simulink model "generic_src"  (Simulink 10.3)
settings: Solver=ode45  StartTime=0.0  StopTime=inf  RelTol=1e-3  EnableMultiTasking=on
undefined symbols (not defined in the file or in its folder): Area_Front, Area_Rear, ay_max_off, ay_max_on, ay_per_mu_max_off, ay_per_mu_max_on, Brake_ratio, brake_valve_ctrl_kP, cat1mode1_higher, cat1mode1_lower, cat1mode2_higher, cat1mode2_lower, cat1mode3_higher, cat1mode3_lower, cat2mode1_higher, cat2mode1_lower, cat2mode2_higher, cat2mode2_lower, cat2mode3_higher, cat2mode3_lower, delta_vel, diff_lock_fac, diff_lock_off, diff_lock_on, ESP_ctrl_kD, ESP_ctrl_kI, ESP_ctrl_kP, ESP_ctrl_restore_kI, ESP_min_throttle_fac, f_ax, f_slip, g, higherlimit_highvel, higherlimit_lowvel, highervel_fac, highervelocity_fac, InitialConditionForIntegrator, limit_acc, limit_selectlow, limit_starting, limit_vdiff, locktime_throttle, lowerlimit_highvel, lowerlimit_lowvel, lowervel_fac, lowervelocity_fac, min_throttle, MPS2KMPH, MSR_ctrl_kD, MSR_ctrl_kI, MSR_ctrl_kP, MSR_min_throttle_fac, PID_kP_sideslip, PID_kP_yawrate, RADpS2RpM, rBrake, RpM2RADpS, SH_SL_switch, sideslip_vel_corr, sidesplip_deviation_max ... (+35)
libraries: CarMaker4SL x136, simulink x55, simulink_extras x6
(part 8 of 9)

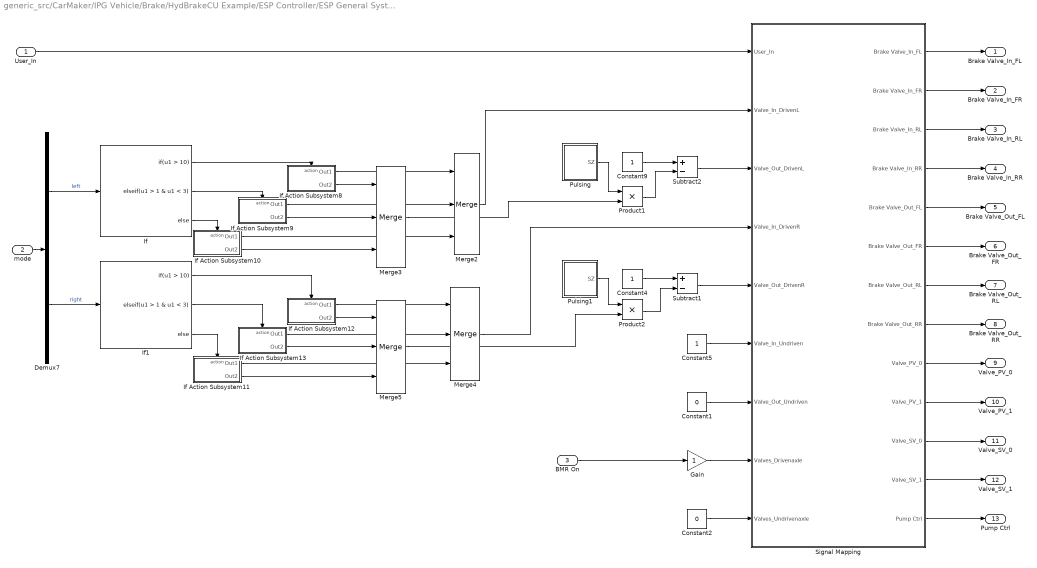
== system generic_src/CarMaker/IPG Vehicle/Brake/HydBrakeCU Example/ESP Controller/ESP General System/ASR/BMR ECU/BMR Controller ==
  User_In : Inport
  mode : Inport  Port=2
  BMR On : Inport  Port=3
  Constant1 : Constant  Value=0
  Constant2 : Constant  Value=0
  Constant4 : Constant
  Constant5 : Constant
  Constant9 : Constant
  Demux7 : Demux  Outputs=2
  Gain : Gain
  If : If  IfExpression=u1 > 10  ElseIfExpressions=u1 > 1 & u1 < 3
  If Action Subsystem10 : Subsystem  TreatAsAtomicUnit=on
  If Action Subsystem11 : Subsystem  TreatAsAtomicUnit=on
  If Action Subsystem12 : Subsystem  TreatAsAtomicUnit=on
  If Action Subsystem13 : Subsystem  TreatAsAtomicUnit=on
  If Action Subsystem8 : Subsystem  TreatAsAtomicUnit=on
  If Action Subsystem9 : Subsystem  TreatAsAtomicUnit=on
  If1 : If  IfExpression=u1 > 10  ElseIfExpressions=u1 > 1 & u1 < 3
  Merge{2..5} (4 alike) : Merge  Inputs=3
  Product1 : Product  RndMeth=Zero
  Product2 : Product  RndMeth=Zero
  Pulsing : Subsystem
  Pulsing1 : Subsystem
  Signal Mapping : Subsystem
  Subtract1 : Sum  Inputs=+-
  Subtract2 : Sum  Inputs=+-
  Brake Valve_In_FL : Outport  VectorParamsAs1DForOutWhenUnconnected=off
  Brake Valve_In_FR : Outport  Port=2  VectorParamsAs1DForOutWhenUnconnected=off
  Brake Valve_In_RL : Outport  Port=3  VectorParamsAs1DForOutWhenUnconnected=off
  Brake Valve_In_RR : Outport  Port=4  VectorParamsAs1DForOutWhenUnconnected=off
  Brake Valve_Out_FL : Outport  Port=5  VectorParamsAs1DForOutWhenUnconnected=off
  Brake Valve_Out_FR : Outport  Port=6  VectorParamsAs1DForOutWhenUnconnected=off
  Brake Valve_Out_RL : Outport  Port=7  VectorParamsAs1DForOutWhenUnconnected=off
  Brake Valve_Out_RR : Outport  Port=8  VectorParamsAs1DForOutWhenUnconnected=off
  Valve_PV_0 : Outport  Port=9  VectorParamsAs1DForOutWhenUnconnected=off
  Valve_PV_1 : Outport  Port=10  VectorParamsAs1DForOutWhenUnconnected=off
  Valve_SV_0 : Outport  Port=11  VectorParamsAs1DForOutWhenUnconnected=off
  Valve_SV_1 : Outport  Port=12  VectorParamsAs1DForOutWhenUnconnected=off
  Pump Ctrl : Outport  Port=13  VectorParamsAs1DForOutWhenUnconnected=off
  wires:
  Demux7/1 -> If/1  "left"
  If/1 -> If Action Subsystem8/Action
  If/2 -> If Action Subsystem9/Action
  If/3 -> If Action Subsystem10/Action
  If Action Subsystem8/1(Out1) -> Merge2/1
  If Action Subsystem9/1(Out1) -> Merge2/2
  If Action Subsystem10/1(Out1) -> Merge2/3
  If Action Subsystem8/2(Out2) -> Merge3/1
  If Action Subsystem9/2(Out2) -> Merge3/2
  If Action Subsystem10/2(Out2) -> Merge3/3
  If1/1 -> If Action Subsystem12/Action
  If1/2 -> If Action Subsystem13/Action
  If1/3 -> If Action Subsystem11/Action
  If Action Subsystem12/1(Out1) -> Merge4/1
  If Action Subsystem13/1(Out1) -> Merge4/2
  If Action Subsystem11/1(Out1) -> Merge4/3
  If Action Subsystem12/2(Out2) -> Merge5/1
  If Action Subsystem13/2(Out2) -> Merge5/2
  If Action Subsystem11/2(Out2) -> Merge5/3
  Demux7/2 -> If1/1  "right"
  Merge3/1 -> Product1/2
  Merge5/1 -> Product2/2
  Constant4/1 -> Subtract1/1
  Product2/1 -> Subtract1/2
  Constant9/1 -> Subtract2/1
  Product1/1 -> Subtract2/2
  BMR On/1 -> Gain/1
  mode/1 -> Demux7/1
  Merge2/1 -> Signal Mapping/2(Valve_In_DrivenL)
  Merge4/1 -> Signal Mapping/4(Valve_In_DrivenR)
  Constant5/1 -> Signal Mapping/6(Valve_In_Undriven)
  Constant1/1 -> Signal Mapping/7(Valve_Out_Undriven)
  Gain/1 -> Signal Mapping/8(Valves_Drivenaxle)
  Constant2/1 -> Signal Mapping/9(Valves_Undrivenaxle)
  Signal Mapping/1(Brake Valve_In_FL) -> Brake Valve_In_FL/1
  Signal Mapping/2(Brake Valve_In_FR) -> Brake Valve_In_FR/1
  Signal Mapping/3(Brake Valve_In_RL) -> Brake Valve_In_RL/1
  Signal Mapping/4(Brake Valve_In_RR) -> Brake Valve_In_RR/1
  Signal Mapping/5(Brake Valve_Out_FL) -> Brake Valve_Out_FL/1
  Signal Mapping/6(Brake Valve_Out_FR) -> Brake Valve_Out_FR/1
  Signal Mapping/7(Brake Valve_Out_RL) -> Brake Valve_Out_RL/1
  Signal Mapping/8(Brake Valve_Out_RR) -> Brake Valve_Out_RR/1
  Signal Mapping/9(Valve_PV_0) -> Valve_PV_0/1
  Signal Mapping/10(Valve_PV_1) -> Valve_PV_1/1
  Signal Mapping/11(Valve_SV_0) -> Valve_SV_0/1
  Signal Mapping/12(Valve_SV_1) -> Valve_SV_1/1
  Signal Mapping/13(Pump Ctrl) -> Pump Ctrl/1
  User_In/1 -> Signal Mapping/1(User_In)
  Subtract1/1 -> Signal Mapping/5(Valve_Out_DrivenR)
  Subtract2/1 -> Signal Mapping/3(Valve_Out_DrivenL)
  Pulsing1/1(SZ) -> Product2/1
  Pulsing/1(SZ) -> Product1/1

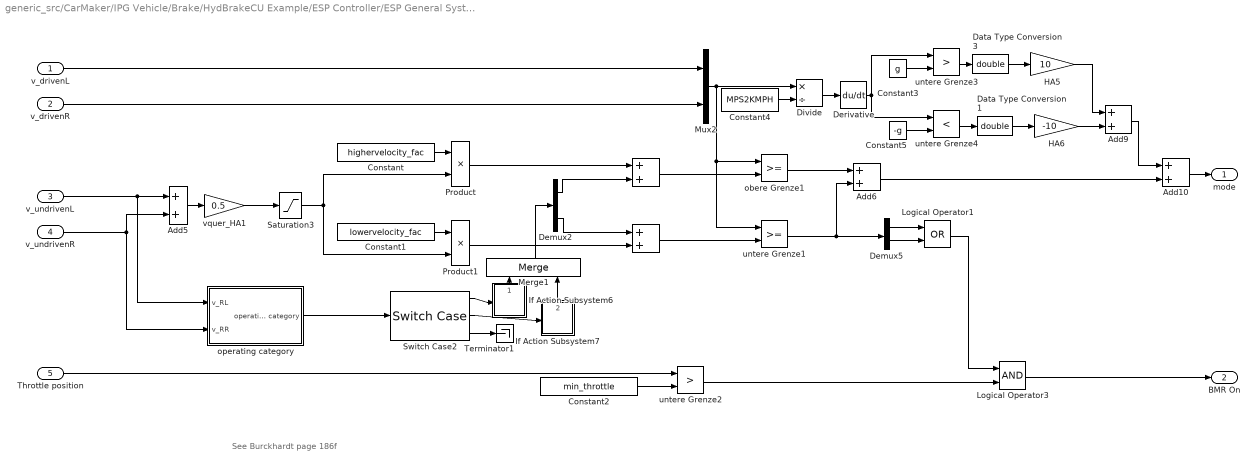
== system generic_src/CarMaker/IPG Vehicle/Brake/HydBrakeCU Example/ESP Controller/ESP General System/ASR/BMR ECU/BMR logic ==
  note: See Burckhardt page 186f
  v_drivenL : Inport
  v_drivenR : Inport  Port=2
  v_undrivenL : Inport  Port=3
  v_undrivenR : Inport  Port=4
  Throttle position : Inport  Port=5
  " " : Sum
  "   " : Sum
  Add{5..6,9..10} (4 alike) : Sum
  Constant : Constant  Value=highervelocity_fac
  Constant1 : Constant  Value=lowervelocity_fac
  Constant2 : Constant  Value=min_throttle
  Constant3 : Constant  Value=g
  Constant4 : Constant  Value=MPS2KMPH
  Constant5 : Constant  Value=-g
  Data Type Conversion1 : DataTypeConversion  OutDataTypeStr=double
  Data Type Conversion3 : DataTypeConversion  OutDataTypeStr=double
  Demux2 : Demux  Outputs=2
  Demux5 : Demux  Outputs=2
  Derivative : Derivative
  Divide : Product  Inputs=*/
  HA5 : Gain  Gain=10
  HA6 : Gain  Gain=-10
  If Action Subsystem6 : Subsystem  TreatAsAtomicUnit=on
  If Action Subsystem7 : Subsystem  TreatAsAtomicUnit=on
  Logical Operator1 : Logic  Operator=OR  AllPortsSameDT=off
  Logical Operator3 : Logic  AllPortsSameDT=off
  Merge1 : Merge
  Mux2 : Mux  Inputs=2
  Product : Product  RndMeth=Zero
  Product1 : Product  RndMeth=Zero
  Saturation3 : Saturate  UpperLimit=inf  LowerLimit=1
  Switch Case2 : SwitchCase  CaseConditions={1,2}
  Terminator1 : Terminator
  obere Grenze1 : RelationalOperator  OutDataTypeStr=boolean  RndMeth=Nearest
  operating category : Subsystem
  untere Grenze1 : RelationalOperator  OutDataTypeStr=boolean  RndMeth=Nearest
  untere Grenze2 : RelationalOperator  Operator=>  RndMeth=Nearest
  untere Grenze3 : RelationalOperator  Operator=>  RndMeth=Nearest
  untere Grenze4 : RelationalOperator  Operator=<  RndMeth=Nearest
  vquer_HA1 : Gain  Gain=0.5
  mode : Outport  VectorParamsAs1DForOutWhenUnconnected=off
  BMR On : Outport  Port=2  VectorParamsAs1DForOutWhenUnconnected=off
  wires:
  Switch Case2/3 -> Terminator1/1
  operating category/1(operating category) -> Switch Case2/1
  Switch Case2/1 -> If Action Subsystem6/Action
  Switch Case2/2 -> If Action Subsystem7/Action
  Merge1/1 -> Demux2/1
  If Action Subsystem6/1(1) -> Merge1/1
  If Action Subsystem7/1(2) -> Merge1/2
  Demux2/1 -> "   "/2
  Add5/1 -> vquer_HA1/1
  vquer_HA1/1 -> Saturation3/1
  Saturation3/1 -> Product1/2, Product/2
  Product/1 -> "   "/1
  Product1/1 -> " "/2
  Demux2/2 -> " "/1
  "   "/1 -> obere Grenze1/2
  obere Grenze1/1 -> Add6/1
  untere Grenze1/1 -> Add6/2, Demux5/1
  untere Grenze3/1 -> Data Type Conversion3/1
  untere Grenze4/1 -> Data Type Conversion1/1
  HA5/1 -> Add9/1
  HA6/1 -> Add9/2
  Data Type Conversion3/1 -> HA5/1
  Data Type Conversion1/1 -> HA6/1
  Derivative/1 -> untere Grenze4/1, untere Grenze3/1
  Add6/1 -> Add10/2
  Divide/1 -> Derivative/1
  Add9/1 -> Add10/1
  Add10/1 -> mode/1
  Demux5/1 -> Logical Operator1/1
  Demux5/2 -> Logical Operator1/2
  Logical Operator3/1 -> BMR On/1
  Throttle position/1 -> untere Grenze2/1
  Logical Operator1/1 -> Logical Operator3/1
  untere Grenze2/1 -> Logical Operator3/2
  v_undrivenL/1 -> operating category/1(v_RL), Add5/1
  v_undrivenR/1 -> Add5/2, operating category/2(v_RR)
  Constant/1 -> Product/1
  Constant1/1 -> Product1/1
  Constant2/1 -> untere Grenze2/2
  Constant4/1 -> Divide/2
  Constant3/1 -> untere Grenze3/2
  Constant5/1 -> untere Grenze4/2
  " "/1 -> untere Grenze1/2
  Mux2/1 -> Divide/1, obere Grenze1/1, untere Grenze1/1
  v_drivenR/1 -> Mux2/2
  v_drivenL/1 -> Mux2/1

== system generic_src/CarMaker/IPG Vehicle/Brake/HydBrakeCU Example/ESP Controller/ESP General System/ASR/BMR ECU/Differential Lock ==
  User_In : Inport
  v_DrivenL : Inport  Port=2
  v_DrivenR : Inport  Port=3
  Abs : Abs
  Add1 : Sum  Inputs=+-
  Bus Selector1 : BusSelector  OutputSignals=User_DiffLock.User_DiffLock_Trq,User_DiffLock.User_DiffLock_on
  Bus Selector2 : BusSelector  OutputSignals=User_Drive
  Constant : Constant  Value=0
  Constant1 : Constant  Value=0
  Constant2 : Constant  Value=diff_lock_fac
  Demux : Demux  Outputs=2
  Mux : Mux  Inputs=2
  Mux1 : Mux  Inputs=2
  Mux2 : Mux  Inputs=2
  Product : Product  RndMeth=Zero
  Relay : Relay  OnSwitchValue=diff_lock_on  OffSwitchValue=diff_lock_off
  Switch1 : Switch  Criteria=u2 > Threshold
  Switch2 : Switch  Criteria=u2 > Threshold  Threshold=1.5
  Switch3 : Switch  Criteria=u2 > Threshold  Threshold=2.5
  Transfer Fcn : TransferFcn  Denominator=[0.1 1]
  FrontDiff_Torque : Outport  VectorParamsAs1DForOutWhenUnconnected=off
  RearDiff_Torque : Outport  Port=2  VectorParamsAs1DForOutWhenUnconnected=off
  wires:
  Abs/1 -> Relay/1
  Relay/1 -> Product/1
  Add1/1 -> Abs/1
  Product/1 -> Transfer Fcn/1
  v_DrivenL/1 -> Add1/1
  v_DrivenR/1 -> Add1/2
  User_In/1 -> Bus Selector2/1, Bus Selector1/1
  Bus Selector2/1 -> Switch2/2, Switch3/2  "<User_Drive>"
  Demux/1 -> FrontDiff_Torque/1
  Demux/2 -> RearDiff_Torque/1
  Switch3/1 -> Demux/1
  Transfer Fcn/1 -> Switch1/3
  Mux/1 -> Switch3/1
  Constant/1 -> Mux1/1
  Mux1/1 -> Switch2/1
  Switch2/1 -> Switch3/3
  Constant1/1 -> Mux2/2
  Mux2/1 -> Switch2/3
  Bus Selector1/2 -> Switch1/2  "<User_DiffLock_on>"
  Bus Selector1/1 -> Switch1/1  "<User_DiffLock_Trq>"
  Switch1/1 -> Mux2/1, Mux1/2, Mux/1, Mux/2
  Constant2/1 -> Product/2

== system generic_src/CarMaker/IPG Vehicle/Brake/HydBrakeCU Example/ESP Controller/ESP General System/ASR/BMR ECU/Signal Mapping ==
  User_In : Inport
  WheelVelocity : Inport  Port=2
  Ideal_In : Inport  Port=3
  Bus Selector1 : BusSelector  OutputSignals=Ideal_Velocity.Ideal_Velocity
  Bus Selector2 : BusSelector  OutputSignals=User_Drive
  Demux1 : Demux
  Demux2 : Demux
  Mux1 : Mux
  Mux2 : Mux
  Mux3 : Mux
  Switch2 : Switch  Criteria=u2 > Threshold  Threshold=1.5
  Switch3 : Switch  Criteria=u2 > Threshold  Threshold=2.5
  v_DrivenL : Outport  VectorParamsAs1DForOutWhenUnconnected=off
  v_DrivenR : Outport  Port=2  VectorParamsAs1DForOutWhenUnconnected=off
  v_UndrivenL : Outport  Port=3  VectorParamsAs1DForOutWhenUnconnected=off
  v_UndrivenR : Outport  Port=4  VectorParamsAs1DForOutWhenUnconnected=off
  wires:
  WheelVelocity/1 -> Demux1/1
  User_In/1 -> Bus Selector2/1
  Bus Selector2/1 -> Switch3/2, Switch2/2  "<User_Drive>"
  Bus Selector1/1 -> Mux3/3, Mux3/4  "<Ideal_Velocity>"
  Mux3/1 -> Switch3/1
  Switch2/1 -> Switch3/3
  Switch3/1 -> Demux2/1
  Demux1/1 -> Mux1/1, Mux3/1, Mux2/3  "v_FL"
  Demux1/2 -> Mux1/2, Mux2/4, Mux3/2  "v_FR"
  Demux1/3 -> Mux1/3, Mux2/1
  Demux1/4 -> Mux1/4, Mux2/2
  Mux1/1 -> Switch2/3
  Mux2/1 -> Switch2/1
  Demux2/1 -> v_DrivenL/1
  Demux2/2 -> v_DrivenR/1
  Demux2/3 -> v_UndrivenL/1
  Demux2/4 -> v_UndrivenR/1
  Ideal_In/1 -> Bus Selector1/1

== system generic_src/CarMaker/IPG Vehicle/Brake/HydBrakeCU Example/ESP Controller/ESP General System/ASR/MSR ECU/MSR logic ==
  v_drivenL : Inport
  v_drivenR : Inport  Port=2
  v_undrivenL : Inport  Port=3
  v_undrivenR : Inport  Port=4
  " " : Gain  Gain=0.5
  "   " : Gain  Gain=0.5
  Add{,1..4} (5 alike) : Sum
  Compare To Zero : simulink/Logic and Bit Operations/Compare To Zero  relop===  OutDataTypeStr=uint8
  Constant : Constant  Value=highervel_fac
  Constant1 : Constant  Value=lowervel_fac
  Demux1 : Demux  Outputs=2
  If Action Subsystem : Subsystem  TreatAsAtomicUnit=on
  If Action Subsystem1 : Subsystem  TreatAsAtomicUnit=on
  If Action Subsystem2 : Subsystem  TreatAsAtomicUnit=on
  If Action Subsystem3 : Subsystem  TreatAsAtomicUnit=on
  If Action Subsystem4 : Subsystem  TreatAsAtomicUnit=on
  If Action Subsystem5 : Subsystem  TreatAsAtomicUnit=on
  Logical Operator : Logic  AllPortsSameDT=off  OutDataTypeStr=boolean
  Merge : Merge  Inputs=6
  Product : Product  RndMeth=Zero
  Product1 : Product  RndMeth=Zero
  Saturation1 : Saturate  UpperLimit=inf  LowerLimit=1
  Saturation2 : Saturate  UpperLimit=inf  LowerLimit=1
  Subtract : Sum  Inputs=+-
  Subtract3 : Sum  Inputs=+-
  Switch Case1 : SwitchCase  CaseConditions={11,12,13,21,22,23}
  Terminator : Terminator
  lower bound : RelationalOperator  OutDataTypeStr=boolean  RndMeth=Nearest
  operating category : Subsystem
  operating mode : Subsystem
  upper bound : RelationalOperator  OutDataTypeStr=boolean  RndMeth=Nearest
  Pseudo_slip : Outport  VectorParamsAs1DForOutWhenUnconnected=off
  reduce torque : Outport  Port=2  VectorParamsAs1DForOutWhenUnconnected=off
  hold torque : Outport  Port=3  VectorParamsAs1DForOutWhenUnconnected=off
  wires:
  Add1/1 -> " "/1
  Add/1 -> "   "/1
  "   "/1 -> Saturation2/1
  " "/1 -> Saturation1/1
  Product/1 -> Add4/1
  operating mode/1(mode) -> Add3/1
  operating category/1(category) -> Add3/2
  Add3/1 -> Switch Case1/1
  Switch Case1/1 -> If Action Subsystem/Action
  Merge/1 -> Demux1/1
  Switch Case1/2 -> If Action Subsystem1/Action
  Switch Case1/3 -> If Action Subsystem2/Action
  Switch Case1/4 -> If Action Subsystem3/Action
  Switch Case1/5 -> If Action Subsystem4/Action
  Switch Case1/6 -> If Action Subsystem5/Action
  If Action Subsystem/1(1.1) -> Merge/1
  If Action Subsystem1/1(1.2) -> Merge/2
  If Action Subsystem2/1(1.3) -> Merge/3
  If Action Subsystem3/1(2.1) -> Merge/4
  If Action Subsystem4/1(2.2) -> Merge/5
  If Action Subsystem5/1(2.3) -> Merge/6
  Switch Case1/7 -> Terminator/1
  Demux1/1 -> Add4/2
  Add2/1 -> lower bound/2, Subtract3/2
  upper bound/1 -> reduce torque/1, Compare To Zero/1  "reduce moment flag"
  lower bound/1 -> Logical Operator/2
  Compare To Zero/1 -> Logical Operator/1
  Logical Operator/1 -> hold torque/1  "hold moment flag"
  Subtract/1 -> upper bound/1, lower bound/1, Subtract3/1
  Saturation1/1 -> Subtract/1
  Saturation2/1 -> Product1/1, Subtract/2, Product/2
  Add4/1 -> upper bound/2
  Subtract3/1 -> Pseudo_slip/1
  Demux1/2 -> Add2/1
  Product1/1 -> Add2/2
  v_drivenL/1 -> operating category/1(v_drivenL), Add1/1
  v_drivenR/1 -> operating category/2(v_drivenR), Add1/2
  v_undrivenR/1 -> operating category/4(v_undrivenR), operating mode/2(v_undrivenR), Add/2
  v_undrivenL/1 -> operating category/3(v_undrivenL), operating mode/1(v_undrivenL), Add/1
  Constant/1 -> Product/1
  Constant1/1 -> Product1/2

== system generic_src/CarMaker/IPG Vehicle/Brake/HydBrakeCU Example/ESP Controller/ESP General System/ASR/MSR ECU/MSR/Gas Controller ==
  Throttle_position : Inport
  Pseudo_Slip : Inport  Port=2
  close Gas : Inport  Port=3
  hold Gas : Inport  Port=4
  Compare To Zero : simulink/Logic and Bit Operations/Compare To Zero  relop===  OutDataTypeStr=uint8
  Constant1 : Constant  Value=MSR_min_throttle_fac
  Constant2 : Constant  Value=min_throttle
  Data Type Conversion2 : DataTypeConversion
  Enabled Subsystem : Subsystem  TreatAsAtomicUnit=on
  Logical Operator : Logic  Operator=OR  AllPortsSameDT=off
  Logical Operator1 : Logic  AllPortsSameDT=off
  PID Controller : Subsystem
  Product2 : Product  SaturateOnIntegerOverflow=on  OutDataTypeStr=Inherit: Same as first input
  Saturation Dynamic : simulink/Discontinuities/Saturation Dynamic  OutMin=[]  OutMax=[]  OutDataTypeStr=Inherit: Same as second input  OutDataType=sfix(16)  OutScaling=2^-10  DoSatur=off
  Subtract : Sum  Inputs=-+
  Switch1 : Switch  Criteria=u2 > Threshold  Threshold=0.5
  Switch3 : Switch  Criteria=u2 > Threshold
  untere Grenze2 : RelationalOperator  Operator=>  RndMeth=Nearest
  vquer_VA1 : Gain
  MSR_On : Outport  VectorParamsAs1DForOutWhenUnconnected=off
  Gas_Out : Outport  Port=2  VectorParamsAs1DForOutWhenUnconnected=off
  wires:
  hold Gas/1 -> Enabled Subsystem/Trigger, Logical Operator/2, Switch1/2
  Switch3/1 -> Switch1/3, Enabled Subsystem/1(In1)
  Compare To Zero/1 -> Data Type Conversion2/1
  close Gas/1 -> Logical Operator/1, Compare To Zero/1, Switch3/2
  Data Type Conversion2/1 -> PID Controller/2(RESET)
  Enabled Subsystem/1(Out1) -> Switch1/1
  Switch1/1 -> Gas_Out/1
  Throttle_position/1 -> Switch3/3, Product2/1, vquer_VA1/1, Subtract/2, untere Grenze2/1
  PID Controller/1(y) -> Subtract/1
  Pseudo_Slip/1 -> PID Controller/1(u)
  Saturation Dynamic/1 -> Switch3/1
  vquer_VA1/1 -> Saturation Dynamic/1
  Product2/1 -> Saturation Dynamic/3
  Subtract/1 -> Saturation Dynamic/2
  Constant1/1 -> Product2/2
  Constant2/1 -> untere Grenze2/2
  untere Grenze2/1 -> Logical Operator1/2
  Logical Operator/1 -> Logical Operator1/1
  Logical Operator1/1 -> MSR_On/1

== system generic_src/CarMaker/IPG Vehicle/Brake/HydBrakeCU Example/ESP Controller/ESP General System/ASR/MSR ECU/Signal Mapping ==
  WheelVelocity : Inport
  User_In : Inport  Port=2
  Ideal_In : Inport  Port=3
  Bus Selector1 : BusSelector  OutputSignals=Ideal_Velocity.Ideal_Velocity
  Bus Selector2 : BusSelector  OutputSignals=User_Drive
  Demux : Demux
  Demux2 : Demux
  Mux1 : Mux
  Mux2 : Mux
  Mux3 : Mux
  Switch2 : Switch  Criteria=u2 > Threshold  Threshold=1.5
  Switch3 : Switch  Criteria=u2 > Threshold  Threshold=2.5
  v_DrivenL : Outport  VectorParamsAs1DForOutWhenUnconnected=off
  v_DrivenR : Outport  Port=2  VectorParamsAs1DForOutWhenUnconnected=off
  v_UndrivenL : Outport  Port=3  VectorParamsAs1DForOutWhenUnconnected=off
  v_UndrivenR : Outport  Port=4  VectorParamsAs1DForOutWhenUnconnected=off
  wires:
  WheelVelocity/1 -> Demux/1
  User_In/1 -> Bus Selector2/1
  Bus Selector2/1 -> Switch3/2, Switch2/2  "<User_Drive>"
  Mux3/1 -> Switch3/1
  Switch2/1 -> Switch3/3
  Switch3/1 -> Demux2/1
  Demux/1 -> Mux1/1, Mux3/1, Mux2/3  "v_FL"
  Demux/2 -> Mux1/2, Mux2/4, Mux3/2  "v_FR"
  Demux/3 -> Mux1/3, Mux2/1
  Demux/4 -> Mux1/4, Mux2/2
  Mux1/1 -> Switch2/3
  Mux2/1 -> Switch2/1
  Demux2/1 -> v_DrivenL/1
  Demux2/2 -> v_DrivenR/1
  Demux2/3 -> v_UndrivenL/1
  Demux2/4 -> v_UndrivenR/1
  Bus Selector1/1 -> Mux3/4, Mux3/3  "<Ideal_Velocity>"
  Ideal_In/1 -> Bus Selector1/1

== system generic_src/CarMaker/IPG Vehicle/Brake/HydBrakeCU Example/ESP Controller/ESP General System/ESP/Actuator Brake/pressure distribution target ==
  note: comes from the used brake model
  Trq Out FL : Inport
  Trq Out FR : Inport  Port=2
  Trq Out RL : Inport  Port=3
  Trq Out RR : Inport  Port=4
  Area_Front : Constant  Value=Area_Front
  Area_Rear : Constant  Value=Area_Rear
  Product{1..3,5} (4 alike) : Product  Inputs=*/  RndMeth=Zero
  Product4 : Product  Inputs=***  RndMeth=Zero
  Product6 : Product  Inputs=***  RndMeth=Zero
  rBrake : Constant  Value=rBrake
  ratio : Constant  Value=Brake_ratio
  brake pressure FL : Outport  VectorParamsAs1DForOutWhenUnconnected=off
  brake pressure FR : Outport  Port=2  VectorParamsAs1DForOutWhenUnconnected=off
  brake pressure RL : Outport  Port=3  VectorParamsAs1DForOutWhenUnconnected=off
  brake pressure RR : Outport  Port=4  VectorParamsAs1DForOutWhenUnconnected=off
  wires:
  Trq Out FL/1 -> Product5/1
  Trq Out FR/1 -> Product1/1
  Trq Out RL/1 -> Product2/1
  Trq Out RR/1 -> Product3/1
  Product4/1 -> Product1/2, Product5/2
  Product6/1 -> Product2/2, Product3/2
  Product5/1 -> brake pressure FL/1
  Product1/1 -> brake pressure FR/1
  Product2/1 -> brake pressure RL/1
  Product3/1 -> brake pressure RR/1
  Area_Front/1 -> Product4/1
  rBrake/1 -> Product4/2, Product6/1
  ratio/1 -> Product4/3, Product6/2
  Area_Rear/1 -> Product6/3

== system generic_src/CarMaker/IPG Vehicle/Brake/HydBrakeCU Example/ESP Controller/ESP General System/ESP/Actuator Brake/pressure reallocation ==
  target_pressure_FL : Inport
  target_pressure_FR : Inport  Port=2
  target_pressure_RL : Inport  Port=3
  target_pressure_RR : Inport  Port=4
  actual_pressure_FL : Inport  Port=5
  actual_pressure_FR : Inport  Port=6
  actual_pressure_RL : Inport  Port=7
  actual_pressure_RR : Inport  Port=8
  Add{,1..3} (4 alike) : Sum
  Compare To Zero{,1..3} (4 alike) : simulink/Logic and Bit Operations/Compare To Zero  relop=<  OutDataTypeStr=uint8
  Data Type Conversion{,1..3} (4 alike) : DataTypeConversion
  Gain{,1..3} (4 alike) : Gain  Gain=-1
  Logical Operator{,1..3} (4 alike) : Logic  AllPortsSameDT=off  OutDataTypeStr=boolean
  Mux : Mux
  Mux1 : Mux
  Product{,1..3} (4 alike) : Product  RndMeth=Zero
  Relational Operator{,1..3} (4 alike) : RelationalOperator  Operator=<  OutDataTypeStr=boolean  RndMeth=Nearest
  Subtract : Sum  Inputs=+-
  Pressure deviation : Outport  VectorParamsAs1DForOutWhenUnconnected=off
  wires:
  Subtract/1 -> Pressure deviation/1
  Mux/1 -> Subtract/2  "ist"
  target_pressure_FL/1 -> Add1/2, Product/1, Relational Operator/1, Compare To Zero/1
  Mux1/1 -> Subtract/1  "soll"
  actual_pressure_FR/1 -> Relational Operator1/2, Mux/2
  actual_pressure_RL/1 -> Relational Operator2/2, Mux/3
  actual_pressure_FL/1 -> Mux/1, Relational Operator/2
  actual_pressure_RR/1 -> Relational Operator3/2, Mux/4
  Compare To Zero/1 -> Logical Operator/1
  Relational Operator/1 -> Logical Operator/2
  Compare To Zero1/1 -> Logical Operator1/1
  Relational Operator1/1 -> Logical Operator1/2
  Compare To Zero2/1 -> Logical Operator2/1
  Relational Operator2/1 -> Logical Operator2/2
  Compare To Zero3/1 -> Logical Operator3/1
  Relational Operator3/1 -> Logical Operator3/2
  Logical Operator/1 -> Data Type Conversion/1
  Gain/1 -> Product/2
  target_pressure_FR/1 -> Product1/1, Relational Operator1/1, Compare To Zero1/1, Add/2
  Logical Operator1/1 -> Data Type Conversion1/1
  Gain1/1 -> Product1/2
  target_pressure_RL/1 -> Add3/2, Product2/1, Relational Operator2/1, Compare To Zero2/1
  Logical Operator2/1 -> Data Type Conversion2/1
  Gain2/1 -> Product2/2
  target_pressure_RR/1 -> Compare To Zero3/1, Relational Operator3/1, Product3/1, Add2/2
  Logical Operator3/1 -> Data Type Conversion3/1
  Gain3/1 -> Product3/2
  Product/1 -> Add/1
  Product1/1 -> Add1/1
  Add1/1 -> Mux1/1
  Add/1 -> Mux1/2
  Product2/1 -> Add2/1
  Add2/1 -> Mux1/4
  Product3/1 -> Add3/1
  Add3/1 -> Mux1/3
  Data Type Conversion/1 -> Gain/1
  Data Type Conversion1/1 -> Gain1/1
  Data Type Conversion2/1 -> Gain2/1
  Data Type Conversion3/1 -> Gain3/1

== system generic_src/CarMaker/IPG Vehicle/Brake/HydBrakeCU Example/ESP Controller/ESP General System/ESP/ECU/ECU logic ==
  note: The ON/OFF relay blocks can be modified
      | in order to delay the trigger of the ESC
  SideSlipAngle deviation : Inport
  YawRate corrected deviation : Inport  Port=2
  mu_max : Inport  Port=3
  Ideal_In : Inport  Port=4
  "    " : Constant  Value=yawrate_vel_corr
  "         " : Constant  Value=sideslip_vel_corr
  Bus Selector1 : BusSelector  OutputSignals=Ideal_Velocity.Ideal_Velocity
  Dead Zone : DeadZone  LowerValue=-0.001  UpperValue=0.001  SaturateOnIntegerOverflow=on
  Dead Zone1 : DeadZone  LowerValue=-0.001  UpperValue=0.001  SaturateOnIntegerOverflow=on
  Define CM Dict3 : CarMaker4SL/Define CM Dict  xname=ESP.ESP_Stabilizing_torque  xunit=Nm  xmono=off  xtype=Double4  xdvaplace=None  xnstates=0  xfirststate=0  xinitial=0
  ON/OFF : Relay  OnSwitchValue=0  OffSwitchValue=0  ZeroCross=off
  ON/OFF1 : Relay  OnSwitchValue=0  OffSwitchValue=0  ZeroCross=off
  P Slip angle : Subsystem
  P Yaw Rate : Subsystem
  "SideSlipAngle : maximum authorized deviation" : Constant  Value=sidesplip_deviation_max
  Sign : Relay  OnSwitchValue=0  OffSwitchValue=0  OffOutputValue=-1
  Sign1 : Relay  OnSwitchValue=0  OffSwitchValue=0  OffOutputValue=-1
  Sum1 : Sum  Inputs=|+-  InputSameDT=on  SaturateOnIntegerOverflow=on  OutDataTypeStr=Inherit: Same as first input
  Sum3 : Sum  Inputs=|+-  InputSameDT=on  SaturateOnIntegerOverflow=on  OutDataTypeStr=Inherit: Same as first input
  Sum5 : Sum  Inputs=-+  InputSameDT=on  SaturateOnIntegerOverflow=on  OutDataTypeStr=Inherit: Same as first input
  Sum6 : Sum  Inputs=+-  InputSameDT=on  SaturateOnIntegerOverflow=on  OutDataTypeStr=Inherit: Same as first input
  Sum8 : Sum  Inputs=+-  InputSameDT=on  SaturateOnIntegerOverflow=on  OutDataTypeStr=Inherit: Same as first input
  Threshold correction coefficient  as regards vehicle's velocity : Subsystem
  Write CM Dict3 : CarMaker4SL/Write CM Dict  xname=ESP.ESP_Stabilizing_torque  xsync=off
  "YawRate : maximum authorized corrected deviation" : Constant  Value=yawrate_deviation_max
  epsilon1 : Product  Inputs=**
  epsilon10 : Product  Inputs=*/
  epsilon{2,4..9,13..15} (10 alike) : Product
  epsilon3 : Product  Inputs=**
  shut down ESP if v<v lim : Subsystem
  v lim : Constant  Value=v_min
  v lim (in m/s) : Constant  Value=MPS2KMPH
  Stabilizing Torque : Outport  VectorParamsAs1DForOutWhenUnconnected=off
  wires:
  Sum3/1 -> P Slip angle/1(x), epsilon1/1
  SideSlipAngle deviation/1 -> Dead Zone/1, Sum3/1
  Sign/1 -> epsilon8/2, epsilon1/2
  epsilon8/1 -> Sum3/2
  Dead Zone/1 -> Sign/1
  epsilon1/1 -> ON/OFF/1
  Sum1/1 -> P Yaw Rate/1(x), epsilon3/1
  YawRate corrected deviation/1 -> Sum1/1, Dead Zone1/1
  Sign1/1 -> epsilon4/2, epsilon3/2
  epsilon4/1 -> Sum1/2
  Dead Zone1/1 -> Sign1/1
  epsilon3/1 -> ON/OFF1/1
  ON/OFF/1 -> epsilon5/2
  ON/OFF1/1 -> epsilon6/2
  epsilon9/1 -> Stabilizing Torque/1, Write CM Dict3/1
  shut down ESP if v<v lim/1(ON/OFF velocity condition) -> epsilon9/2
  epsilon6/1 -> Sum5/2
  epsilon5/1 -> Sum5/1
  Sum5/1 -> epsilon9/1
  epsilon14/1 -> Sum6/2
  epsilon13/1 -> Sum8/2
  Threshold correction coefficient  as regards vehicle's velocity/1(Threshold correction coefficient) -> epsilon2/2
  mu_max/1 -> epsilon2/1, Sum6/1, Sum8/1
  Sum8/1 -> epsilon15/2
  epsilon15/1 -> epsilon8/1
  "SideSlipAngle : maximum authorized deviation"/1 -> epsilon15/1
  epsilon2/1 -> epsilon13/2, epsilon14/1
  "YawRate : maximum authorized corrected deviation"/1 -> epsilon7/1
  Sum6/1 -> epsilon7/2
  epsilon7/1 -> epsilon4/1
  Bus Selector1/1 -> Threshold correction coefficient  as regards vehicle's velocity/1(v), shut down ESP if v<v lim/1(v)  "<Ideal_Velocity>"
  Ideal_In/1 -> Bus Selector1/1
  v lim (in m/s)/1 -> epsilon10/2
  v lim/1 -> epsilon10/1
  epsilon10/1 -> shut down ESP if v<v lim/2(v lim ESP)
  P Slip angle/1(y) -> epsilon5/1
  P Yaw Rate/1(y1) -> epsilon6/1
  "    "/1 -> epsilon14/2
  "         "/1 -> epsilon13/1

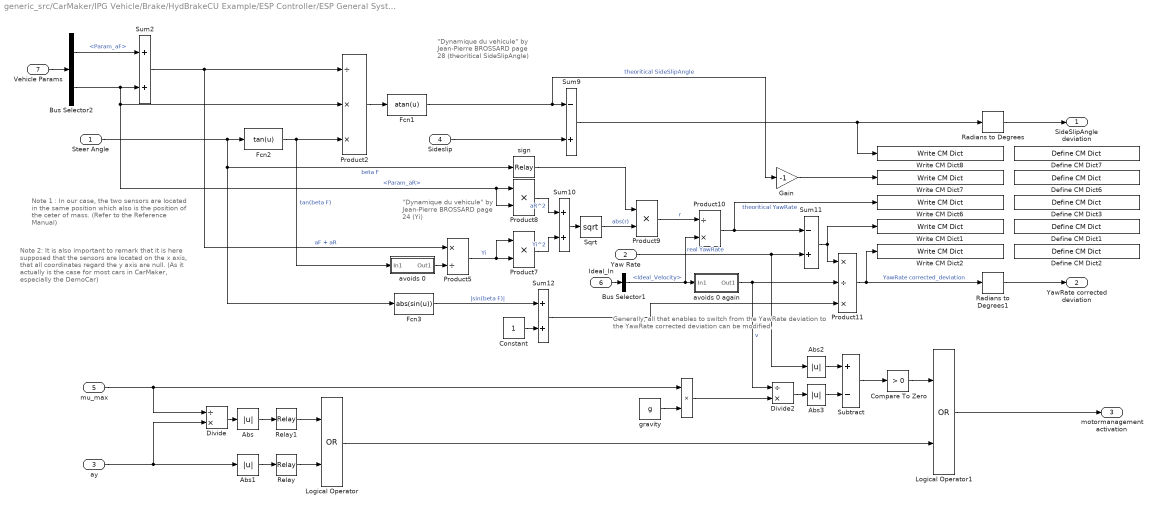
== system generic_src/CarMaker/IPG Vehicle/Brake/HydBrakeCU Example/ESP Controller/ESP General System/ESP/ECU/Instability detectors ==
  note: Note 1 :
      | In our case, the two sensors
      | are located in the same position
      | which also is the position of the ceter of mass.
      | (Refer to the Reference Manual)
  note: Note 2:
      | It is also important to remark that it is here
      | supposed that the sensors are located on the x axis,
      | that all coordinates regard the y axis are null.
      | (As it actually is the case for most cars in CarMaker,
      | especially the DemoCar)
  note: "Dynamique du vehicule"
      | by Jean-Pierre BROSSARD
      | page 28
      | (theoritical SideSlipAngle)
  note: Generally, all that enables to switch from the YawRate deviation
      | to the YawRate corrected deviation can be modified.
  note: "Dynamique du vehicule"
      | by Jean-Pierre BROSSARD
      | page 24
      | (Yi)
  Steer Angle : Inport
  Yaw Rate : Inport  Port=2
  ay : Inport  Port=3
  Sideslip : Inport  Port=4
  mu_max : Inport  Port=5
  Ideal_In : Inport  Port=6
  Vehicle Params : Inport  Port=7
  " " : Product  Inputs=**
  Abs{,1..3} (4 alike) : Abs
  Bus Selector1 : BusSelector  OutputSignals=Ideal_Velocity.Ideal_Velocity
  Bus Selector2 : BusSelector  OutputSignals=VehicleGeometry.Param_aF,VehicleGeometry.Param_aR
  Compare To Zero : simulink/Logic and Bit Operations/Compare To Zero  relop=>  OutDataTypeStr=uint8
  Constant : Constant
  Define CM Dict1 : CarMaker4SL/Define CM Dict  xname=ESP.YawRate_deviation  xunit=rad/s  xmono=off  xtype=Double4  xdvaplace=None  xnstates=0  xfirststate=0  xinitial=0
  Define CM Dict2 : CarMaker4SL/Define CM Dict  xname=ESP.YawRate_corrected_deviation  xunit=rad/m  xmono=off  xtype=Double4  xdvaplace=None  xnstates=0  xfirststate=0  xinitial=0
  Define CM Dict3 : CarMaker4SL/Define CM Dict  xname=ESP.YawRate_theoretical  xunit=rad/s  xmono=off  xtype=Double4  xdvaplace=None  xnstates=0  xfirststate=0  xinitial=0
  Define CM Dict6 : CarMaker4SL/Define CM Dict  xname=ESP.SideSlipeAngle_theoretical  xunit=rad  xmono=off  xtype=Double4  xdvaplace=None  xnstates=0  xfirststate=0  xinitial=0
  Define CM Dict7 : CarMaker4SL/Define CM Dict  xname=ESP.SideSlipAngle_deviation  xunit=rad  xmono=off  xtype=Double4  xdvaplace=None  xnstates=0  xfirststate=0  xinitial=0
  Divide : Product  Inputs=/*
  Divide2 : Product  Inputs=/*
  Fcn1 : Fcn  Expr=atan(u)
  Fcn2 : Fcn  Expr=tan(u)
  Fcn3 : Fcn  Expr=abs(sin(u))
  Gain : Gain  Gain=-1
  Logical Operator : Logic  Operator=OR  AllPortsSameDT=off  OutDataTypeStr=boolean
  Logical Operator1 : Logic  Operator=OR  AllPortsSameDT=off  OutDataTypeStr=boolean
  Product10 : Product  Inputs=/*  RndMeth=Zero
  Product11 : Product  Inputs=*/*  RndMeth=Zero
  Product2 : Product  Inputs=/**  RndMeth=Zero
  Product5 : Product  Inputs=*/  RndMeth=Zero
  Product7 : Product  RndMeth=Zero
  Product8 : Product  RndMeth=Zero
  Product9 : Product  RndMeth=Zero
  Radians to Degrees : simulink_extras/Transformations/Radians to Degrees
  Radians to Degrees1 : simulink_extras/Transformations/Radians to Degrees
  Relay : Relay  OnSwitchValue=ay_max_on  OffSwitchValue=ay_max_off
  Relay1 : Relay  OnSwitchValue=ay_per_mu_max_on  OffSwitchValue=ay_per_mu_max_off
  Sqrt : Math  Operator=sqrt  SignedPower=on  SaturateOnIntegerOverflow=on
  Subtract : Sum  Inputs=+-
  Sum10 : Sum  Inputs=2  InputSameDT=on  SaturateOnIntegerOverflow=on  OutDataTypeStr=Inherit: Same as first input
  Sum11 : Sum  Inputs=-+  InputSameDT=on  SaturateOnIntegerOverflow=on  OutDataTypeStr=Inherit: Same as first input
  Sum12 : Sum  InputSameDT=on  SaturateOnIntegerOverflow=on  OutDataTypeStr=Inherit: Same as first input
  Sum2 : Sum  Inputs=2  InputSameDT=on  SaturateOnIntegerOverflow=on  OutDataTypeStr=Inherit: Same as first input
  Sum9 : Sum  Inputs=-+  InputSameDT=on  SaturateOnIntegerOverflow=on  OutDataTypeStr=Inherit: Same as first input
  Write CM Dict1 : CarMaker4SL/Write CM Dict  xname=ESP.YawRate_deviation  xsync=off
  Write CM Dict2 : CarMaker4SL/Write CM Dict  xname=ESP.YawRate_corrected_deviation  xsync=off
  Write CM Dict6 : CarMaker4SL/Write CM Dict  xname=ESP.YawRate_theoretical  xsync=off
  Write CM Dict7 : CarMaker4SL/Write CM Dict  xname=ESP.SideSlipeAngle_theoretical  xsync=off
  Write CM Dict8 : CarMaker4SL/Write CM Dict  xname=ESP.SideSlipAngle_deviation  xsync=off
  avoids 0 : Subsystem
  avoids 0 again : Subsystem
  gravity : Constant  Value=g
  sign : Relay  OnSwitchValue=0  OffSwitchValue=0  OffOutputValue=-1
  SideSlipAngle deviation : Outport  VectorParamsAs1DForOutWhenUnconnected=off
  YawRate corrected deviation : Outport  Port=2  VectorParamsAs1DForOutWhenUnconnected=off
  motormanagement activation : Outport  Port=3  VectorParamsAs1DForOutWhenUnconnected=off
  wires:
  Steer Angle/1 -> Fcn2/1, sign/1, Fcn3/1  "beta F"
  Bus Selector2/1 -> Sum2/1  "<Param_aF>"
  Bus Selector2/2 -> Product8/1, Product8/2, Product2/2, Sum2/2  "<Param_aR>"
  Fcn2/1 -> avoids 0/1(In1), Product2/3  "tan(beta F)"
  Sum2/1 -> Product5/1, Product2/1  "aF + aR"
  Sum9/1 -> Radians to Degrees/1, Write CM Dict8/1
  Product2/1 -> Fcn1/1
  Fcn1/1 -> Sum9/1, Gain/1  "theoritical SideSlipAngle"
  Sideslip/1 -> Sum9/2
  Product5/1 -> Product7/2, Product7/1  "Yi"
  Product8/1 -> Sum10/1  "aR^2"
  Product7/1 -> Sum10/2  "Yi^2"
  Sum10/1 -> Sqrt/1
  Sqrt/1 -> Product9/2  "abs(r)"
  sign/1 -> Product9/1
  avoids 0/1(Out1) -> Product5/2
  Product9/1 -> Product10/1  "r"
  Product10/1 -> Sum11/1, Write CM Dict6/1  "theoritical YawRate"
  Yaw Rate/1 -> Sum11/2, Abs2/1  "real YawRate"
  Bus Selector1/1 -> Product10/2, avoids 0 again/1(In1)  "<Ideal_Velocity>"
  Constant/1 -> Sum12/2
  Product11/1 -> Radians to Degrees1/1, Write CM Dict2/1  "YawRate corrected_deviation"
  Sum11/1 -> Product11/1, Write CM Dict1/1
  Fcn3/1 -> Sum12/1  "|sin(beta F)|"
  avoids 0 again/1(Out1) -> Divide2/1, Product11/2  "v"
  Radians to Degrees/1 -> SideSlipAngle deviation/1
  Radians to Degrees1/1 -> YawRate corrected deviation/1
  Sum12/1 -> Product11/3
  Divide/1 -> Abs/1
  Abs/1 -> Relay1/1
  Abs1/1 -> Relay/1
  ay/1 -> Divide/2, Abs1/1
  mu_max/1 -> Divide/1, " "/1
  gravity/1 -> " "/2
  " "/1 -> Divide2/2
  Divide2/1 -> Abs3/1
  Abs2/1 -> Subtract/1
  Abs3/1 -> Subtract/2
  Subtract/1 -> Compare To Zero/1
  Logical Operator1/1 -> motormanagement activation/1
  Compare To Zero/1 -> Logical Operator1/1
  Logical Operator/1 -> Logical Operator1/2
  Relay1/1 -> Logical Operator/1
  Relay/1 -> Logical Operator/2
  Ideal_In/1 -> Bus Selector1/1
  Vehicle Params/1 -> Bus Selector2/1
  Gain/1 -> Write CM Dict7/1

== system generic_src/CarMaker/IPG Vehicle/Brake/HydBrakeCU Example/ESP Controller/ESP General System/ESP/ECU/Motor management strategy ==
  activation DK : Inport
  Throttle_position : Inport  Port=2
  ax : Inport  Port=3
  Abs1 : Abs
  Compare To Zero : simulink/Logic and Bit Operations/Compare To Zero  relop===  OutDataTypeStr=uint8
  Constant : Constant  Value=ESP_min_throttle_fac
  Data Type Conversion2 : DataTypeConversion
  PID-Controller : Subsystem
  Product : Product  RndMeth=Zero
  Saturation Dynamic : simulink/Discontinuities/Saturation Dynamic  OutMin=[]  OutMax=[]  OutDataTypeStr=Inherit: Same as second input  OutDataType=sfix(16)  OutScaling=2^-10  DoSatur=off
  Switch1 : Switch  Criteria=u2 > Threshold
  Switch3 : Switch  Criteria=u2 > Threshold
  restoration to driver : Subsystem
  vquer_VA1 : Gain
  Gas_out : Outport  VectorParamsAs1DForOutWhenUnconnected=off
  wires:
  Compare To Zero/1 -> Data Type Conversion2/1
  Data Type Conversion2/1 -> PID-Controller/2(RESET)
  Throttle_position/1 -> Switch3/3, Product/1, vquer_VA1/1
  vquer_VA1/1 -> Saturation Dynamic/1
  Product/1 -> Saturation Dynamic/3
  activation DK/1 -> Compare To Zero/1, Switch3/2, restoration to driver/2(activation on)
  PID-Controller/1(y) -> Saturation Dynamic/2
  Saturation Dynamic/1 -> Switch3/1, restoration to driver/1(controller in)
  Switch3/1 -> Switch1/3, restoration to driver/3(driver in)
  Switch1/1 -> Gas_out/1
  restoration to driver/1(Control Gas) -> Switch1/1
  ax/1 -> Abs1/1
  Abs1/1 -> PID-Controller/1(u)
  restoration to driver/2(restoration) -> Switch1/2
  Constant/1 -> Product/2

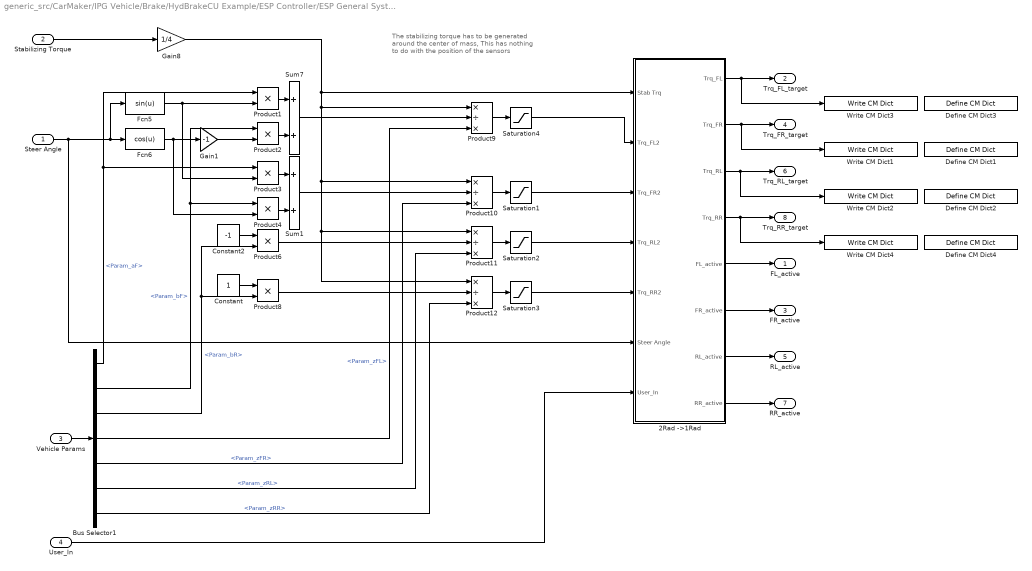
== system generic_src/CarMaker/IPG Vehicle/Brake/HydBrakeCU Example/ESP Controller/ESP General System/ESP/ECU/brake distribution strategy ==
  note: The stabilizing torque has to be generated
      | around the center of mass,
      | This has nothing to do with
      | the position of the sensors
  Steer Angle : Inport
  Stabilizing Torque : Inport  Port=2
  Vehicle Params : Inport  Port=3
  User_In : Inport  Port=4
  2Rad ->1Rad : Subsystem
  Bus Selector1 : BusSelector  OutputSignals=VehicleGeometry.Param_aF,VehicleGeometry.Param_bF,VehicleGeometry.Param_bR,CarrierGeometry.Param_zFL,CarrierGeometry.Param_zFR,CarrierGeometry.Param_zRL,CarrierGeometry.Param_zRR
  Constant : Constant
  Constant2 : Constant  Value=-1
  Define CM Dict1 : CarMaker4SL/Define CM Dict  xname=ESP.ESP_corr_Trq_FR  xunit=Nm  xmono=off  xtype=Double4  xdvaplace=None  xnstates=0  xfirststate=0  xinitial=0
  Define CM Dict2 : CarMaker4SL/Define CM Dict  xname=ESP.ESP_corr_Trq_RL  xunit=Nm  xmono=off  xtype=Double4  xdvaplace=None  xnstates=0  xfirststate=0  xinitial=0
  Define CM Dict3 : CarMaker4SL/Define CM Dict  xname=ESP.ESP_corr_Trq_FL  xunit=Nm  xmono=off  xtype=Double4  xdvaplace=None  xnstates=0  xfirststate=0  xinitial=0
  Define CM Dict4 : CarMaker4SL/Define CM Dict  xname=ESP.ESP_corr_Trq_RR  xunit=Nm  xmono=off  xtype=Double4  xdvaplace=None  xnstates=0  xfirststate=0  xinitial=0
  Fcn5 : Fcn  Expr=sin(u)
  Fcn6 : Fcn  Expr=cos(u)
  Gain1 : Gain  Gain=-1
  Gain8 : Gain  Gain=1/4
  Product{1..4,6,8} (6 alike) : Product  RndMeth=Zero
  Product{9..12} (4 alike) : Product  Inputs=*/*  RndMeth=Zero
  Saturation{1..4} (4 alike) : Saturate  UpperLimit=3000  LowerLimit=-3000
  Sum1 : Sum  Inputs=2  InputSameDT=on  SaturateOnIntegerOverflow=on  OutDataTypeStr=Inherit: Same as first input
  Sum7 : Sum  Inputs=2  InputSameDT=on  SaturateOnIntegerOverflow=on  OutDataTypeStr=Inherit: Same as first input
  Write CM Dict1 : CarMaker4SL/Write CM Dict  xname=ESP.ESP_corr_Trq_FR  xsync=off
  Write CM Dict2 : CarMaker4SL/Write CM Dict  xname=ESP.ESP_corr_Trq_RL  xsync=off
  Write CM Dict3 : CarMaker4SL/Write CM Dict  xname=ESP.ESP_corr_Trq_FL  xsync=off
  Write CM Dict4 : CarMaker4SL/Write CM Dict  xname=ESP.ESP_corr_Trq_RR  xsync=off
  FL_active : Outport  VectorParamsAs1DForOutWhenUnconnected=off
  Trq_FL_target : Outport  Port=2  VectorParamsAs1DForOutWhenUnconnected=off
  FR_active : Outport  Port=3  VectorParamsAs1DForOutWhenUnconnected=off
  Trq_FR_target : Outport  Port=4  VectorParamsAs1DForOutWhenUnconnected=off
  RL_active : Outport  Port=5  VectorParamsAs1DForOutWhenUnconnected=off
  Trq_RL_target : Outport  Port=6  VectorParamsAs1DForOutWhenUnconnected=off
  RR_active : Outport  Port=7  VectorParamsAs1DForOutWhenUnconnected=off
  Trq_RR_target : Outport  Port=8  VectorParamsAs1DForOutWhenUnconnected=off
  wires:
  Steer Angle/1 -> Fcn5/1, Fcn6/1, 2Rad ->1Rad/6(Steer Angle)
  Fcn5/1 -> Product1/2, Product3/2
  Fcn6/1 -> Product4/2, Gain1/1
  Gain1/1 -> Product2/2
  Product1/1 -> Sum7/1
  Product2/1 -> Sum7/2
  Product3/1 -> Sum1/1
  Product4/1 -> Sum1/2
  Product6/1 -> Product11/2
  Product8/1 -> Product12/2
  Sum1/1 -> Product10/2
  Sum7/1 -> Product9/2
  Product9/1 -> Saturation4/1
  Saturation4/1 -> 2Rad ->1Rad/2(Trq_FL2)
  Saturation1/1 -> 2Rad ->1Rad/3(Trq_FR2)
  Saturation3/1 -> 2Rad ->1Rad/5(Trq_RR2)
  Saturation2/1 -> 2Rad ->1Rad/4(Trq_RL2)
  Stabilizing Torque/1 -> Gain8/1
  Gain8/1 -> Product12/1, Product11/1, Product10/1, Product9/1, 2Rad ->1Rad/1(Stab Trq)
  Product10/1 -> Saturation1/1
  Product12/1 -> Saturation3/1
  Product11/1 -> Saturation2/1
  Bus Selector1/3 -> Product6/2, Product8/2  "<Param_bR>"
  Bus Selector1/2 -> Product4/1, Product2/1  "<Param_bF>"
  2Rad ->1Rad/2(Trq_FR) -> Write CM Dict1/1, Trq_FR_target/1
  2Rad ->1Rad/3(Trq_RL) -> Write CM Dict2/1, Trq_RL_target/1
  2Rad ->1Rad/4(Trq_RR) -> Trq_RR_target/1, Write CM Dict4/1
  2Rad ->1Rad/5(FL_active) -> FL_active/1
  2Rad ->1Rad/6(FR_active) -> FR_active/1
  2Rad ->1Rad/7(RL_active) -> RL_active/1
  2Rad ->1Rad/8(RR_active) -> RR_active/1
  Vehicle Params/1 -> Bus Selector1/1
  Bus Selector1/1 -> Product3/1, Product1/1  "<Param_aF>"
  Constant2/1 -> Product6/1
  Constant/1 -> Product8/1
  Bus Selector1/4 -> Product9/3  "<Param_zFL>"
  Bus Selector1/5 -> Product10/3  "<Param_zFR>"
  Bus Selector1/6 -> Product11/3  "<Param_zRL>"
  Bus Selector1/7 -> Product12/3  "<Param_zRR>"
  User_In/1 -> 2Rad ->1Rad/7(User_In)
  2Rad ->1Rad/1(Trq_FL) -> Write CM Dict3/1, Trq_FL_target/1

== system generic_src/CarMaker/IPG Vehicle/Brake/HydBrakeCU Example/ESP Controller/ESP General System/ESP/helpsignals estimator/SideSlip estimator ==
  lenkwinkel : Inport
  CarMaker_In : Inport  Port=2
  Bus Selector1 : BusSelector  OutputSignals=Ideal_Velocity.Ideal_Velocity_y,Ideal_Velocity.Ideal_Velocity_x
  Constant1 : Constant  Value=0
  Divide6 : Product  Inputs=*/
  Switch : Switch  Threshold=1
  Terminator : Terminator
  Trigonometric Function2 : Trigonometry  Operator=atan
  SideSlipAngle_estimated : Outport  VectorParamsAs1DForOutWhenUnconnected=off
  wires:
  Bus Selector1/2 -> Divide6/2, Switch/2  "<Ideal_Velocity_x>"
  Divide6/1 -> Trigonometric Function2/1
  Trigonometric Function2/1 -> Switch/1
  Constant1/1 -> Switch/3
  Switch/1 -> SideSlipAngle_estimated/1
  lenkwinkel/1 -> Terminator/1
  CarMaker_In/1 -> Bus Selector1/1
  Bus Selector1/1 -> Divide6/1  "<Ideal_Velocity_y>"

== system generic_src/CarMaker/IPG Vehicle/Brake/HydBrakeCU Example/ESP Controller/ESP General System/ESP/helpsignals estimator/mue estimator ==
  CarMaker_In : Inport
  Vehicle Params : Inport  Port=2
  Bus Selector1 : BusSelector  OutputSignals=Idea_Trq2W.Ideal_Trq2WRL,Ideal_Fz.Ideal_FzRL,Ideal_Slip.Ideal_SlipRL,Ideal_Velocity.Ideal_Velocity_x,Ideal_YawRate
  Bus Selector2 : BusSelector  OutputSignals=TireRadius.Param_RadiusRL,TireRadius.Param_RadiusRR
  Bus Selector3 : BusSelector  OutputSignals=Idea_Trq2W.Ideal_Trq2WRR,Ideal_Fz.Ideal_FzRR,Ideal_Slip.Ideal_SlipRR,Ideal_Velocity.Ideal_Velocity_x,Ideal_YawRate
  MinMax : MinMax  Inputs=2
  estimator_RL : Subsystem
  estimator_RR : Subsystem
  mue_estimated : Outport  VectorParamsAs1DForOutWhenUnconnected=off
  wires:
  MinMax/1 -> mue_estimated/1
  estimator_RL/1(mue_est_RL) -> MinMax/1
  estimator_RR/1(mue_est_RR) -> MinMax/2
  CarMaker_In/1 -> Bus Selector3/1, Bus Selector1/1
  Vehicle Params/1 -> Bus Selector2/1
  Bus Selector2/1 -> estimator_RL/6(Radius_RL)  "<Param_RadiusRL>"
  Bus Selector2/2 -> estimator_RR/6(Radius_RR)  "<Param_RadiusRR>"
  Bus Selector1/3 -> estimator_RL/3(LongSlip_RL)  "<Ideal_SlipRL>"
  Bus Selector1/4 -> estimator_RL/4(Car_vx)  "<Ideal_Velocity_x>"
  Bus Selector1/2 -> estimator_RL/2(Fz_RL)  "<Ideal_FzRL>"
  Bus Selector1/5 -> estimator_RL/5(YawRate)  "<Ideal_YawRate>"
  Bus Selector1/1 -> estimator_RL/1(Trq2W_RL)  "<Ideal_Trq2WRL>"
  Bus Selector3/1 -> estimator_RR/1(Trq2W_RR)  "<Ideal_Trq2WRR>"
  Bus Selector3/2 -> estimator_RR/2(Fz_RR)  "<Ideal_FzRR>"
  Bus Selector3/3 -> estimator_RR/3(LongSlip_RR)  "<Ideal_SlipRR>"
  Bus Selector3/4 -> estimator_RR/4(Car_vx)  "<Ideal_Velocity_x>"
  Bus Selector3/5 -> estimator_RR/5(YawRate)  "<Ideal_YawRate>"

== system generic_src/CarMaker/IPG Vehicle/Brake/HydBrakeCU Example/ESP Controller/ESP General System/ABS/ABS ECU/ABS_ValveCtrl_FL/Duty ==
  Constant1 : Constant  Value=1/t_Sensor
  Integrator : Integrator  ExternalReset=either
  Pulse Generator : DiscretePulseGenerator  PulseType=Time based  Period=t_Sensor*2  PulseWidth=50
  SZ : Outport  VectorParamsAs1DForOutWhenUnconnected=off
  wires:
  Pulse Generator/1 -> Integrator/2
  Constant1/1 -> Integrator/1
  Integrator/1 -> SZ/1

== system generic_src/CarMaker/IPG Vehicle/Brake/HydBrakeCU Example/ESP Controller/ESP General System/ABS/ABS ECU/ABS_ValveCtrl_FR/Duty ==
  Constant1 : Constant  Value=1/t_Sensor
  Integrator : Integrator  ExternalReset=either
  Pulse Generator : DiscretePulseGenerator  PulseType=Time based  Period=t_Sensor*2  PulseWidth=50
  SZ : Outport  VectorParamsAs1DForOutWhenUnconnected=off
  wires:
  Integrator/1 -> SZ/1
  Pulse Generator/1 -> Integrator/2
  Constant1/1 -> Integrator/1

== system generic_src/CarMaker/IPG Vehicle/Brake/HydBrakeCU Example/ESP Controller/ESP General System/ABS/ABS ECU/select_low/ABS_ValveCtrl_rear ==
  note: Valve Control:
      | Valves are open for a predefined time window.
      | The driving time depends on a trigger criterion (LUT).
      | The treshold change for the valve driving time is
      | continously modified by a repeating sequence.
  note: EITHER ABS is switched on and  S_K is put through
      |  when S_K is becomming bigger the s_{ku}
      | OR output is 0 when S_K is smaller than {sku}_{off}
  Sk : Inport
  Constant : Constant
  Duty : Subsystem
  Look-Up Table1 : Lookup  InputValues=Valve_LUTin_HA  Table=ValveIn_LUTout_HA  LookUpMeth=Interpolation-Use End Values  SaturateOnIntegerOverflow=on
  Look-Up Table2 : Lookup  InputValues=Valve_LUTin_HA  Table=ValveOut_LUTout_HA  LookUpMeth=Interpolation-Use End Values  SaturateOnIntegerOverflow=on
  Product : Product  SaturateOnIntegerOverflow=on  OutDataTypeStr=Inherit: Same as first input
  Rate Transition{1..4} (4 alike) : RateTransition
  Relational Operator : RelationalOperator  Operator=<  SampleTime=0.001  RndMeth=Nearest
  Relational Operator1 : RelationalOperator  Operator=<  SampleTime=0.001  RndMeth=Nearest
  Relay : Relay  OnSwitchValue=sku_HA  OffSwitchValue=sku_off_HA
  Sum1 : Sum  Inputs=--+  SaturateOnIntegerOverflow=on
  Zero-Order Hold : ZeroOrderHold  SampleTime=t_Sensor
  Brake.Valve.In : Outport  VectorParamsAs1DForOutWhenUnconnected=off
  Brake.Valve.Out : Outport  Port=2  VectorParamsAs1DForOutWhenUnconnected=off
  Brake.ABS.status : Outport  Port=3  VectorParamsAs1DForOutWhenUnconnected=off
  Brake.ABS.on/off : Outport  Port=4  VectorParamsAs1DForOutWhenUnconnected=off
  wires:
  Sk/1 -> Zero-Order Hold/1
  Product/1 -> Look-Up Table1/1, Look-Up Table2/1
  Relay/1 -> Rate Transition4/1, Product/2
  Zero-Order Hold/1 -> Product/1, Relay/1
  Look-Up Table2/1 -> Rate Transition3/1
  Look-Up Table1/1 -> Rate Transition1/1
  Duty/1(SZ) -> Rate Transition2/1
  Sum1/1 -> Brake.ABS.status/1
  Constant/1 -> Sum1/3
  Relational Operator1/1 -> Sum1/2, Brake.Valve.Out/1
  Relational Operator/1 -> Sum1/1, Brake.Valve.In/1
  Rate Transition2/1 -> Relational Operator1/1, Relational Operator/1
  Rate Transition1/1 -> Relational Operator/2
  Rate Transition3/1 -> Relational Operator1/2
  Rate Transition4/1 -> Brake.ABS.on/off/1

== system generic_src/CarMaker/IPG Vehicle/Brake/HydBrakeCU Example/ESP Controller/ESP General System/ASR/BMR ECU/BMR Controller/If Action Subsystem10 ==
  Action Port : ActionPort
  Constant3 : Constant  Value=ValveIn_abbau
  Constant4 : Constant  Value=ValveOut_abbau
  Out1 : Outport  InitialOutput=[ValveIn_abbau]  VectorParamsAs1DForOutWhenUnconnected=off
  Out2 : Outport  Port=2  InitialOutput=[ValveOut_abbau]  VectorParamsAs1DForOutWhenUnconnected=off
  wires:
  Constant3/1 -> Out1/1
  Constant4/1 -> Out2/1

== system generic_src/CarMaker/IPG Vehicle/Brake/HydBrakeCU Example/ESP Controller/ESP General System/ASR/BMR ECU/BMR Controller/If Action Subsystem11 ==
  Action Port : ActionPort
  Constant3 : Constant  Value=ValveIn_abbau
  Constant4 : Constant  Value=ValveOut_abbau
  Out1 : Outport  InitialOutput=[ValveIn_abbau]  VectorParamsAs1DForOutWhenUnconnected=off
  Out2 : Outport  Port=2  InitialOutput=[ValveOut_abbau]  VectorParamsAs1DForOutWhenUnconnected=off
  wires:
  Constant3/1 -> Out1/1
  Constant4/1 -> Out2/1

== system generic_src/CarMaker/IPG Vehicle/Brake/HydBrakeCU Example/ESP Controller/ESP General System/ASR/BMR ECU/BMR Controller/If Action Subsystem12 ==
  Action Port : ActionPort
  Constant2 : Constant  Value=ValveIn_aufbau_long
  Constant3 : Constant  Value=ValveOut_aufbau_long
  Out1 : Outport  InitialOutput=[ValveIn_aufbau_long]  VectorParamsAs1DForOutWhenUnconnected=off
  Out2 : Outport  Port=2  InitialOutput=[ValveOut_aufbau_long]  VectorParamsAs1DForOutWhenUnconnected=off
  wires:
  Constant3/1 -> Out2/1
  Constant2/1 -> Out1/1

== system generic_src/CarMaker/IPG Vehicle/Brake/HydBrakeCU Example/ESP Controller/ESP General System/ASR/BMR ECU/BMR Controller/If Action Subsystem13 ==
  Action Port : ActionPort
  Constant2 : Constant  Value=ValveIn_aufbau_short
  Constant3 : Constant  Value=ValveOut_aufbau_short
  Out1 : Outport  InitialOutput=[ValveIn_aufbau_short]  VectorParamsAs1DForOutWhenUnconnected=off
  Out2 : Outport  Port=2  InitialOutput=[ValveOut_aufbau_short]  VectorParamsAs1DForOutWhenUnconnected=off
  wires:
  Constant2/1 -> Out1/1
  Constant3/1 -> Out2/1

== system generic_src/CarMaker/IPG Vehicle/Brake/HydBrakeCU Example/ESP Controller/ESP General System/ASR/BMR ECU/BMR Controller/If Action Subsystem8 ==
  Action Port : ActionPort
  Constant2 : Constant  Value=ValveIn_aufbau_long
  Constant3 : Constant  Value=ValveOut_aufbau_long
  Out1 : Outport  InitialOutput=[ValveIn_aufbau_long]  VectorParamsAs1DForOutWhenUnconnected=off
  Out2 : Outport  Port=2  InitialOutput=[ValveOut_aufbau_long]  VectorParamsAs1DForOutWhenUnconnected=off
  wires:
  Constant2/1 -> Out1/1
  Constant3/1 -> Out2/1

== system generic_src/CarMaker/IPG Vehicle/Brake/HydBrakeCU Example/ESP Controller/ESP General System/ASR/BMR ECU/BMR Controller/If Action Subsystem9 ==
  Action Port : ActionPort
  Constant2 : Constant  Value=ValveIn_aufbau_short
  Constant3 : Constant  Value=ValveOut_aufbau_short
  Out1 : Outport  InitialOutput=[ValveIn_aufbau_short]  VectorParamsAs1DForOutWhenUnconnected=off
  Out2 : Outport  Port=2  InitialOutput=[ValveOut_aufbau_short]  VectorParamsAs1DForOutWhenUnconnected=off
  wires:
  Constant2/1 -> Out1/1
  Constant3/1 -> Out2/1

== system generic_src/CarMaker/IPG Vehicle/Brake/HydBrakeCU Example/ESP Controller/ESP General System/ASR/BMR ECU/BMR Controller/Pulsing ==
  Constant1 : Constant  Value=1/t_Sensor
  Integrator : Integrator  ExternalReset=either
  Pulse Generator : DiscretePulseGenerator  PulseType=Time based  Period=t_Sensor*2  PulseWidth=50
  SZ : Outport  VectorParamsAs1DForOutWhenUnconnected=off
  wires:
  Pulse Generator/1 -> Integrator/2
  Constant1/1 -> Integrator/1
  Integrator/1 -> SZ/1
